simulink model "furuta_pi_hardware"  (R2026b)
settings: Solver=FixedStepDiscrete  StopTime=inf  FixedStep=0.005  EnableMultiTasking=on
model workspace (MAT data in the model file):
  calibration = [-209.05 -1 4058.5 1]
  drive = [0 0 0 0]
  limits = [0 0 9 0]
libraries: raspberrypiCommlib x5
settings Model: Creator=Lsh  LastModifiedBy=Lsh
settings SolverCC: PositivePriorityOrder=on
settings OptimizationCC: DifferentSizesBufferReuse=on  EfficientTunableParamExpr=on  EnhancedBackFolding=on  MaxStackSize=200000  OptimizationCustomize=off  OptimizeBlockOrder=speed  PassReuseOutputArgsAs=Individual arguments  RemoveInternalMemoryZeroInit=on  RemoveRootLevelIOMemoryZeroInit=on
settings DebuggingCC: ParameterTunabilityLossMsg=error
settings HardwareCC: ProdHWDeviceType=ARM Compatible->ARM Cortex-A (64-bit)  ProdLargestAtomicFloat=Double  ProdLargestAtomicInteger=LongLong  ProdLongLongMode=on
settings RTWCC: BuildConfiguration=Faster Runs  Description=Embedded Coder  HardwareBoard=Raspberry Pi (64bit)  SystemTargetFile=ert.tlc  TLCOptions="-aInlineSetEventsForThisBaseRateFcn=TLC_FALSE -aSuppressMultiTaskScheduler=TLC_FALSE  -aRateBasedStepFcn=0"  TemplateMakefile=ert_default_tmf  Toolchain=GNU GCC RPIUtils
settings CodeAppCC: ForceParamTrailComments=on  IgnoreCustomStorageClasses=off  InsertBlockDesc=on  OperatorAnnotations=on  SFDataObjDesc=on  SimulinkDataObjDesc=on
settings ERTTargetCC: CombineSignalStateStructs=on  ExtModeIntrfLevel=Level2 - Open  ExtModeMexFile=ext_xcp  ExtModeStaticAlloc=on  SupportVariableSizeSignals=on

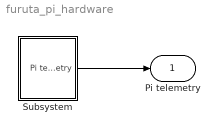
== system furuta_pi_hardware ==
  Subsystem : Subsystem
  Pi telemetry : Outport
  wires:
  Subsystem/1(Pi telemetry) -> Pi telemetry/1

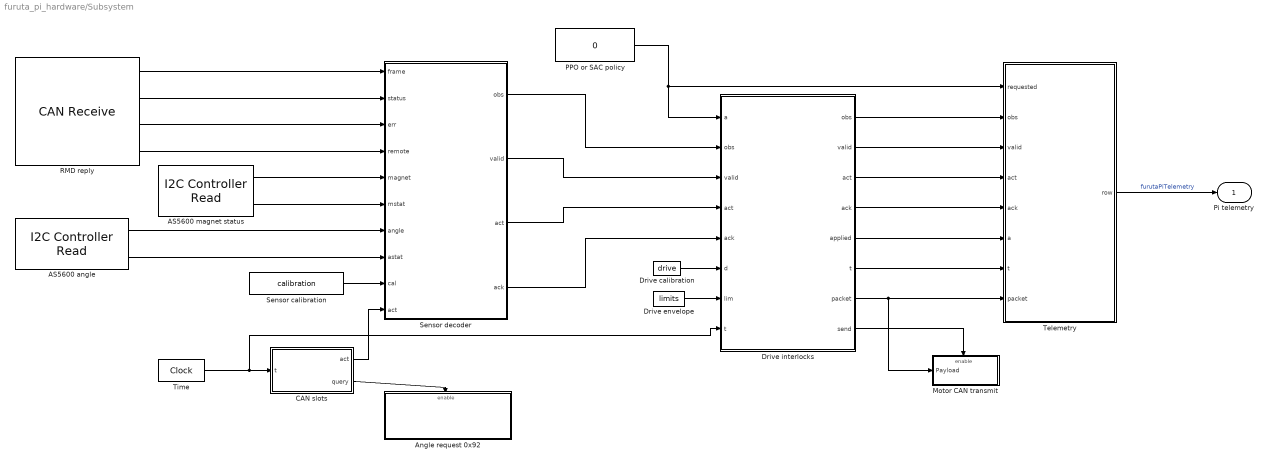
== system furuta_pi_hardware/Subsystem ==
  AS5600 angle : raspberrypiCommlib/I2C Controller Read  BoardProperty=Pi 5 Model  I2CModule=1  Mode=Master  SlaveAddress=54  SlaveByteOrder=BigEndian  Direction=Receiver  RegisterAddressMode=on  RegisterAddress=14  SlaveDataType=uint8  DataLength=2  NoAck=off  RepeatedStart=on  OutputStatus=on  SampleTime=.005
  AS5600 magnet status : raspberrypiCommlib/I2C Controller Read  BoardProperty=Pi 5 Model  I2CModule=1  Mode=Master  SlaveAddress=54  SlaveByteOrder=BigEndian  Direction=Receiver  RegisterAddressMode=on  RegisterAddress=11  SlaveDataType=uint8  DataLength=1  NoAck=off  RepeatedStart=on  OutputStatus=on  SampleTime=.005
  Angle request 0x92 : Subsystem  TreatAsAtomicUnit=on
  CAN slots : MATLAB Function  TreatAsAtomicUnit=on
  Drive calibration : Constant  Value=drive  SampleTime=.005
  Drive envelope : Constant  Value=limits  SampleTime=.005
  Drive interlocks : MATLAB Function  TreatAsAtomicUnit=on
  Motor CAN transmit : Subsystem  TreatAsAtomicUnit=on
  PPO or SAC policy : Constant  Value=0  SampleTime=.005
  RMD reply : raspberrypiCommlib/CAN Receive  DeviceID=can0  SetupCAN=off  TypeofCAN=Real  OutputDataType=Raw data  IdentifierType=Standard (11-bit identifier)  MessageId=577  MsgLength=8  SampleTime=.005  OutputError=on  OutputRemote=on  SimulateUsing=Code generation
  Sensor calibration : Constant  Value=calibration  SampleTime=.005
  Sensor decoder : MATLAB Function  TreatAsAtomicUnit=on
  Telemetry : MATLAB Function  TreatAsAtomicUnit=on
  Time : DigitalClock  SampleTime=.005
  Pi telemetry : Outport
  wires:
  RMD reply/1 -> Sensor decoder/1(frame)
  PPO or SAC policy/1 -> Drive interlocks/1(a), Telemetry/1(requested)
  Drive interlocks/3(act) -> Telemetry/4(act)
  Drive interlocks/1(obs) -> Telemetry/2(obs)
  Drive interlocks/4(ack) -> Telemetry/5(ack)
  Sensor decoder/1(obs) -> Drive interlocks/2("obs ")
  RMD reply/2 -> Sensor decoder/2(status)
  RMD reply/3 -> Sensor decoder/3(err)
  Drive interlocks/2(valid) -> Telemetry/3(valid)
  Sensor decoder/2(valid) -> Drive interlocks/3("valid ")
  RMD reply/4 -> Sensor decoder/4(remote)
  AS5600 magnet status/1 -> Sensor decoder/5(magnet)
  Sensor calibration/1 -> Sensor decoder/9(cal)
  Telemetry/1(row) -> Pi telemetry/1  "furutaPiTelemetry"
  Drive interlocks/7(packet) -> Motor CAN transmit/1(Payload), Telemetry/8(packet)
  AS5600 magnet status/2 -> Sensor decoder/6(mstat)
  Sensor decoder/3(act) -> Drive interlocks/4("act ")
  AS5600 angle/1 -> Sensor decoder/7(angle)
  Drive interlocks/5(applied) -> Telemetry/6(a)
  Time/1 -> CAN slots/1(t), Drive interlocks/8("t ")
  Drive envelope/1 -> Drive interlocks/7(lim)
  AS5600 angle/2 -> Sensor decoder/8(astat)
  CAN slots/2(query) -> Angle request 0x92/Enable
  Drive calibration/1 -> Drive interlocks/6(d)
  Drive interlocks/6(t) -> Telemetry/7(t)
  Sensor decoder/4(ack) -> Drive interlocks/5("ack ")
  CAN slots/1(act) -> Sensor decoder/10("act ")
  Drive interlocks/8(send) -> Motor CAN transmit/Enable

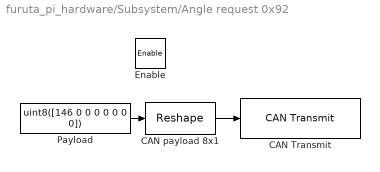
== system furuta_pi_hardware/Subsystem/Angle request 0x92 ==
  Enable : EnablePort
  CAN Transmit : raspberrypiCommlib/CAN Transmit  DeviceID=can0  SetupCAN=off  TypeofCAN=Real  InputDataType=Raw data  BlockingMode_=off  BlockTimeout_=1  OutputStatus=off  IdentifierType=Standard (11-bit identifier)  MessageId=321  MsgLength=8  RemoteFrame=off  SimulateUsing=Code generation
  CAN payload 8x1 : Reshape  OutputDimensionality=Customize  OutputDimensions=[8 1]
  Payload : Constant  Value=uint8([146 0 0 0 0 0 0 0])  SampleTime=.005
  wires:
  Payload/1 -> CAN payload 8x1/1
  CAN payload 8x1/1 -> CAN Transmit/1

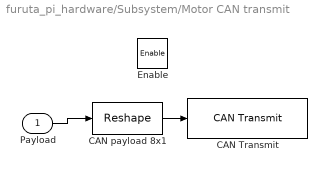
== system furuta_pi_hardware/Subsystem/Motor CAN transmit ==
  Payload : Inport
  Enable : EnablePort
  CAN Transmit : raspberrypiCommlib/CAN Transmit  DeviceID=can0  SetupCAN=off  TypeofCAN=Real  InputDataType=Raw data  BlockingMode_=off  BlockTimeout_=1  OutputStatus=off  IdentifierType=Standard (11-bit identifier)  MessageId=321  MsgLength=8  RemoteFrame=off  SimulateUsing=Code generation
  CAN payload 8x1 : Reshape  OutputDimensionality=Customize  OutputDimensions=[8 1]
  wires:
  Payload/1 -> CAN payload 8x1/1
  CAN payload 8x1/1 -> CAN Transmit/1

== matlab function furuta_pi_hardware/Subsystem/Sensor decoder ==
  data: frame input; obs output; status input; err input; remote input; magnet input; mstat input; angle input; astat input; cal input; act input; valid output; act output; ack output
function [obs,valid,act, ack] = decode(frame,status,err,remote,magnet,mstat,angle,astat,cal,act)
[obs,valid,ack] = furuta_pi_sample(frame,status,err,remote,magnet,mstat,angle,astat,cal,act);
end

== matlab function furuta_pi_hardware/Subsystem/CAN slots ==
  data: act output; t input; query output
function [act, query] = slots(t)
act = mod(round(t/.005),2)==1;
query = ~act;
end

== matlab function furuta_pi_hardware/Subsystem/Drive interlocks ==
  data: obs output; valid output; act output; ack output; applied output; t output; packet output; send output; a input; obs input; valid input; act input; ack input; d input; lim input; t input
function [obs, valid, act, ack,applied, t,packet, send] = command(a,obs,valid,act,ack,d,lim,t)
persistent needsAck count
if isempty(needsAck), needsAck = false; count = 0; end
packet = zeros(1,8,'uint8'); send = false; applied = 0;
if ~act || d(4)==0, return, end
if valid, count = count+1; end
engaged = count>0 || t>.2;
[packet,send,applied] = furuta_pi_frame(a,obs,valid && (~needsAck || ack),engaged,d(1),d(2),d(3),lim,t,d(4));
needsAck = packet(1)==161;

end

== matlab function furuta_pi_hardware/Subsystem/Telemetry ==
  data: requested input; obs input; valid input; act input; ack input; a input; t input; packet input; row output
function row = logrow(requested,obs,valid,act,ack,a,t, packet)
row = [t; double(act); double(valid); obs; a; double(packet(1)); double(ack); requested];
end
